simulink model "TypicalElements"  (R2024b)
settings: Solver=VariableStepAuto  StartTime=0.0  StopTime=10.0  RelTol=1e-3
settings Model: Creator=33242  LastModifiedBy=33242

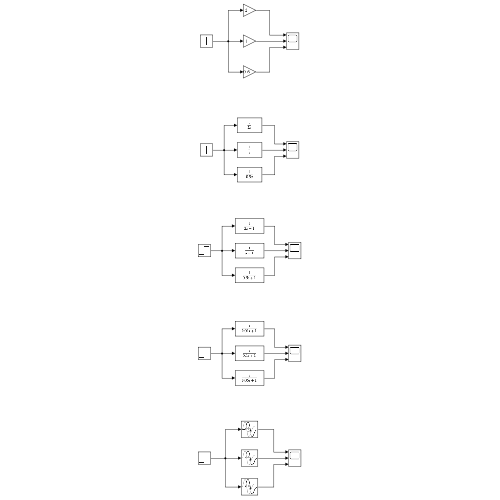
[thumbnail: Simulink's stored preview of the top-level diagram]
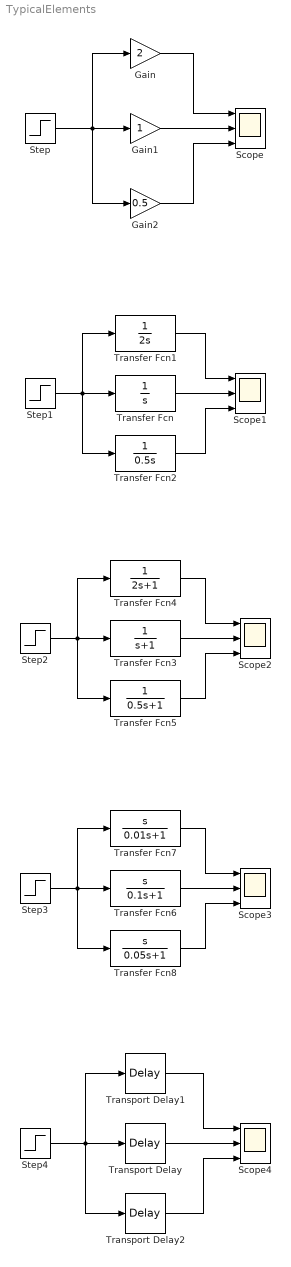
== system TypicalElements ==
  Gain : Gain  Gain=2
  Gain1 : Gain
  Gain2 : Gain  Gain=0.5
  Scope{,1..4} (5 alike) : Scope  NumInputPorts=3
  Step{,1..4} (5 alike) : Step  SampleTime=0
  Transfer Fcn : TransferFcn  Denominator=[1 0]
  Transfer Fcn1 : TransferFcn  Denominator=[2 0]
  Transfer Fcn2 : TransferFcn  Denominator=[0.5 0]
  Transfer Fcn3 : TransferFcn  Denominator=[1 1]
  Transfer Fcn4 : TransferFcn  Denominator=[2 1]
  Transfer Fcn5 : TransferFcn  Denominator=[0.5 1]
  Transfer Fcn6 : TransferFcn  Numerator=[1 0]  Denominator=[0.1 1]
  Transfer Fcn7 : TransferFcn  Numerator=[1 0]  Denominator=[0.01 1]
  Transfer Fcn8 : TransferFcn  Numerator=[1 0]  Denominator=[0.05 1]
  Transport Delay : TransportDelay
  Transport Delay1 : TransportDelay  DelayTime=2
  Transport Delay2 : TransportDelay  DelayTime=0.5
  wires:
  Step/1 -> Gain2/1, Gain/1, Gain1/1
  Gain1/1 -> Scope/2
  Gain/1 -> Scope/1
  Gain2/1 -> Scope/3
  Step1/1 -> Transfer Fcn2/1, Transfer Fcn1/1, Transfer Fcn/1
  Transfer Fcn1/1 -> Scope1/1
  Transfer Fcn/1 -> Scope1/2
  Transfer Fcn2/1 -> Scope1/3
  Transfer Fcn5/1 -> Scope2/3
  Transfer Fcn3/1 -> Scope2/2
  Transfer Fcn4/1 -> Scope2/1
  Step2/1 -> Transfer Fcn3/1, Transfer Fcn4/1, Transfer Fcn5/1
  Step3/1 -> Transfer Fcn8/1, Transfer Fcn7/1, Transfer Fcn6/1
  Transfer Fcn7/1 -> Scope3/1
  Transfer Fcn6/1 -> Scope3/2
  Transfer Fcn8/1 -> Scope3/3
  Step4/1 -> Transport Delay2/1, Transport Delay1/1, Transport Delay/1
  Transport Delay/1 -> Scope4/2
  Transport Delay1/1 -> Scope4/1
  Transport Delay2/1 -> Scope4/3
